simulink model "hrg_wa_compensation_research"  (R2025a)
settings: Solver=FixedStepDiscrete  StartTime=0.0  StopTime=p.duration  FixedStep=p.Ts  RelTol=1e-3
model workspace (MAT data in the model file):
  Ad = [0.987688405123  -5.68131323296e-08  2.48971225508e-05  1.72406495467e-10  2.35500029057e-16  -7.48045553179e-18  2.39085041361e-17  1.59212234261e-22  0  0  0  0; 5.68131323296e-08  0.987688405123  -1.72406495467e-10  2.48971225508e-05  4.70881019476e-18  2.69344781657e-16  -1.59212235008e-22  2.39085041361e-17  0  0  0  0; -982.899001209  -0.00680633562581  0.987672737796  1.37356342331e-05  1.5611837146e-11  -5.09714578103e-13  9.88617178136e-13  1.31942511779e-17  0  0  0  0; 0.00680633562581  -982.899001209  -1.37356342331e-05  0.987672737796  3.12106539235e-13  1.83550880441e-11  -1.31942512097e-17  9.88617178136e-13  0  0  0  0; 0  0  0  0  0.28650479686  0  0  0  0  0  0  0; 0  0  0  0  0  0.352866081459  0  0  0  0  0  0; 943869.866875  6.2854468604  -988.617130951  -0.0131942506432  -1.52887962977e-08  4.97849569843e-10  -9.75634597461e-10  -1.26518662631e-14  0  0  0  0; -6.2854468604  943869.866875  0.0131942506432  -988.617130951  -3.05654153121e-10  -1.79275916498e-08  1.26518662949e-14  -9.75634597462e-10  0  0  0  0; 113668107.931  505.246320907  -239056.237822  -1.59199430864  -2.20191905684e-06  6.98200094534e-08  9.9975990594  -1.46549020767e-12  0.999750031247  0  0  0; -505.246320907  113668107.931  1.59199430864  -239056.237822  -4.4027695682e-08  -2.51395406668e-06  1.46549021355e-12  9.9975990594  0  0.999750031247  0  0; 62170953.3395  1554505.52703  -163920.493963  -4098.88409978  -1.27454644375e-06  4.00156404796e-09  9.50410725413  0.237602681353  0.956612237767  0.0239153059442  0.0432139182638  0; -882829.706009  61193845.2426  2356.91164918  -163353.073245  -7.00440355025e-09  -1.4233603888e-06  -0.139969993764  9.70458623439  -0.0141100303999  0.97829544106  0  0.0591645112941]
  Bd = [1.07541978092e-16  -2.80909408987e-18; 2.15044631223e-18  1.01140599362e-16; 1.17750014529e-11  -3.11685647158e-13; 2.35440509738e-13  1.12226992357e-11; 0.71349520314  0; 0  0.647133918541; -1.10105605369e-08  2.90941885987e-10; -2.20157780066e-10  -1.04757152027e-08; -9.65252715165e-07  2.517993119e-08; -1.93016562843e-08  -9.06591565342e-07; -4.58609339763e-07  1.18833226824e-09; -2.49830556256e-09  -4.18846719335e-07]
  c.detect = [-9972404010.59+545538559.48i  -249313581.813+13639144.7876i; 149497357.356-9010063.9201i  -10364965233+624625194.794i]
  c.sample_period_s = 2.5e-05
  c.drive = [1.0677862215e-06-2.20398678601e-07i  -3.17521221847e-08+7.37459562675e-09i; 2.13558605901e-08-4.40799791844e-09i  1.14308593334e-06-2.65487026279e-07i]
  c.nominal_detect = -9999678898.08+46914376.8426i
  p.schema = 'v10.1'
  p.synthetic = 1
  p.f0 = 1000
  p.gamma_intrinsic = 0.314159265359
  p.Cs = 1e-09
  p.G0 = 1e-10
  p.kappa = 1e-06
  p.b = 1.1e-06
  p.Cds = 0
  p.Rs = 1000
  p.B = 0.276990961962
  p.Omega = 0.5
  p.Ts = 2.5e-05
  p.Tc = 0.001
  p.duration = 0.8
  p.charge_target = 1e-11
  p.initial_fraction = 0.3
  p.theta0 = 0.4
  p.Cf = 1e-10
  p.Rf = 1000000000
  p.driver_tau = [2e-05; 2.4e-05]
  p.afe_bw = [20000; 18000]
  p.detect_matrix = [1  0.025; -0.015  1.04]
  p.drive_matrix = [1  -0.03; 0.02  1.08]
  p.split_hz = 0
  p.stiffness_axis = 0.37
  p.damping_half_difference = 0
  p.damping_axis = -0.23
  p.adc_span = 2
  p.adc_bits = 20
  p.dac_span = 2
  p.dac_bits = 18
  p.vmax = 1
  p.agc_bw = 5
  p.quad_bw = 4
  p.pll_gain = 30
  p.max_detune = 30
  p.virtual_rate = 0
  p.virtual_start_min_s = 0.25
  p.virtual_settle_fraction = 0.01
  p.predict_heading = 1
  p.max_heading_rate = 100
  p.virtual_validated_limit = 0.2
  p.min_amplitude_fraction = 0.02
  p.min_linearity = 0.1
  p.max_calibration_condition = 100
  p.max_frame_age = 0.002
  p.calibrate_detection = 1
  p.calibrate_drive = 1
  p.noise_rms_V = 0
  p.noise_seed = 20261030
  p.heading_start_s = 0
  p.zero_start_force = 1
  p.enable_tensor_ff = 1
  p.identified_dK = [-0.00819482149803  0.00496733694019; 0.00496733694019  0.00671005445861]
  p.identified_dD = [-4.47767757243e-07  -7.60819493737e-07; -7.60819493737e-07  -1.26420490762e-06]
  x0 = [2.76318298201e-12; 1.16825502693e-12; 0; 0; 0; 0; 0; 0; 0; 0; 0; 0]
libraries: hrg_wa_v10_2_cn_modules x5
Description:
  | 条件性补偿研究：合成独立校准参考，原门限不变；20/21研究点通过不等于硬件或全工作范围认证。
settings Model: Creator=11725  LastModifiedBy=11725

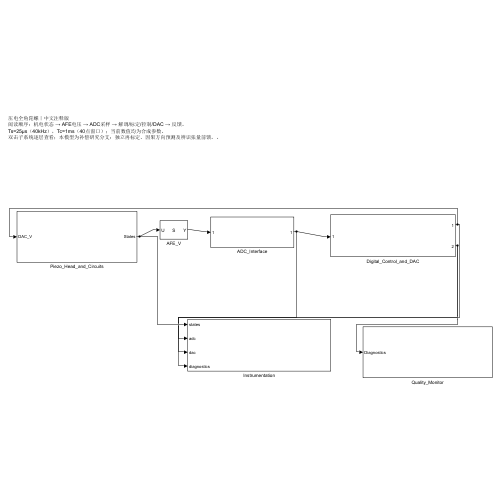
[thumbnail: Simulink's stored preview of the top-level diagram]
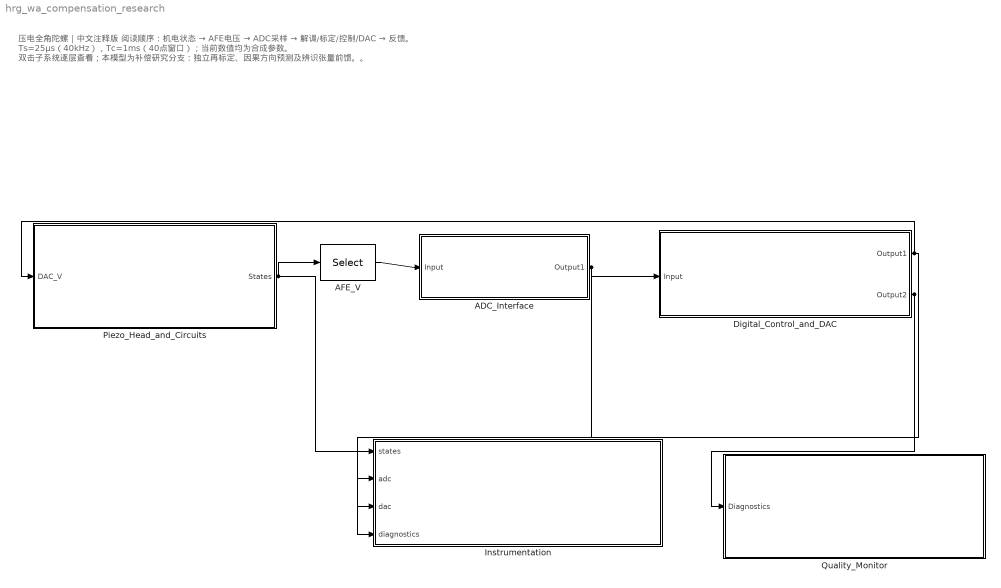
== system hrg_wa_compensation_research ==
  note: 压电全角陀螺｜中文注释版
      | 阅读顺序：机电状态 → AFE电压 → ADC采样 → 解调/标定/控制/DAC → 反馈。
      | Ts=25μs（40kHz），Tc=1ms（40点窗口）；当前数值均为合成参数。
      | 双击子系统逐层查看；本模型为补偿研究分支：独立再标定、因果方向预测及辨识张量前馈。。
  ADC_Interface : Subsystem  Description=输入噪声、ADC整数码量化与两路截幅标志；详见pcn_adc_sfun.m及pcn_quantize.m。
  AFE_V : Selector  InputPortWidth=12  IndexOptions=Index vector (dialog)  Indices=[11 12]  OutputSizes=1
  Digital_Control_and_DAC : Subsystem  Description=补偿研究内核comp_tick：从有效测量开始因果方向预测，首帧前零力；独立辨识ΔK/ΔD前馈。控制不读取真实Omega或机械各向异性真值。
  Instrumentation : Subsystem  Description=14个Scope、2个频谱仪和4组To Workspace；角度评分见pcn_metrics.m。
  Piezo_Head_and_Circuits : Subsystem  Description=压电表头及电路的联合离散模型；五个库模块共12个状态，端口输出顺序见画布。
  Quality_Monitor : Subsystem
  wires:
  Piezo_Head_and_Circuits/1(States) -> AFE_V/1, Instrumentation/1(states)
  AFE_V/1 -> ADC_Interface/1(Input)
  ADC_Interface/1(Output1) -> Digital_Control_and_DAC/1(Input), Instrumentation/2(adc)
  Digital_Control_and_DAC/1(Output1) -> Piezo_Head_and_Circuits/1(DAC_V), Instrumentation/3(dac)
  Digital_Control_and_DAC/2(Output2) -> Instrumentation/4(diagnostics), Quality_Monitor/1(Diagnostics)

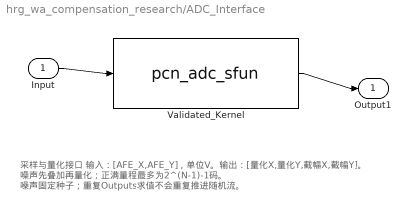
== system hrg_wa_compensation_research/ADC_Interface ==
  note: 采样与量化接口
      | 输入：[AFE_X,AFE_Y]，单位V。输出：[量化X,量化Y,截幅X,截幅Y]。
      | 噪声先叠加再量化；正满量程最多为2^(N-1)-1码。
      | 噪声固定种子；重复Outputs求值不会重复推进随机流。
  Input : Inport
  Validated_Kernel : M-S-Function  FunctionName=pcn_adc_sfun  Parameters=p
  Output1 : Outport
  wires:
  Input/1 -> Validated_Kernel/1
  Validated_Kernel/1 -> Output1/1

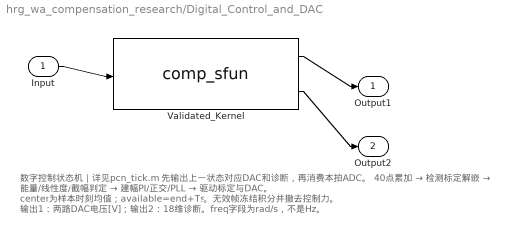
== system hrg_wa_compensation_research/Digital_Control_and_DAC ==
  note: 数字控制状态机｜详见pcn_tick.m
      | 先输出上一状态对应DAC和诊断，再消费本拍ADC。
      | 40点累加 → 检测标定解嵌 → 能量/线性度/截幅判定 → 建幅PI/正交/PLL → 驱动标定与DAC。
      | center为样本时刻均值；available=end+Ts。无效帧冻结积分并撤去控制力。
      | 输出1：两路DAC电压[V]；输出2：18维诊断。freq字段为rad/s，不是Hz。
  Input : Inport
  Validated_Kernel : M-S-Function  Description=comp_sfun调用comp_tick，35维状态不变；前馈为(identified_dK+jω identified_dD)*(I-jQ)，主轴固定在表头坐标。  FunctionName=comp_sfun  Parameters=p,c
  Output1 : Outport
  Output2 : Outport  Port=2
  wires:
  Input/1 -> Validated_Kernel/1
  Validated_Kernel/1 -> Output1/1
  Validated_Kernel/2 -> Output2/1

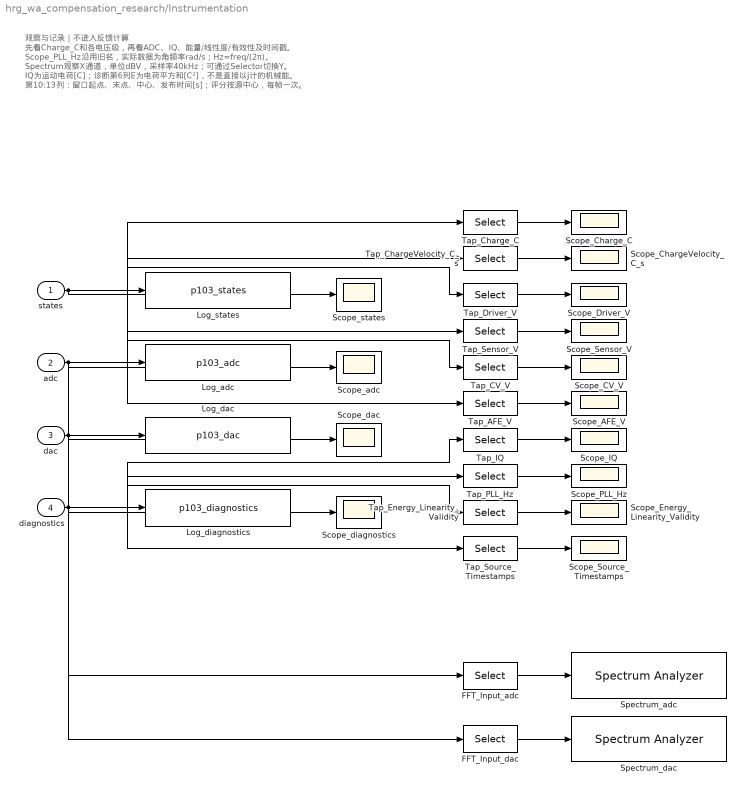
== system hrg_wa_compensation_research/Instrumentation ==
  note: 观察与记录｜不进入反馈计算
      | 先看Charge_C和各电压级，再看ADC、IQ、能量/线性度/有效性及时间戳。
      | Scope_PLL_Hz沿用旧名，实际数据为角频率rad/s；Hz=freq/(2π)。
      | Spectrum观察X通道，单位dBV，采样率40kHz；可通过Selector切换Y。
      | IQ为运动电荷[C]；诊断第6列E为电荷平方和[C²]，不是直接以J计的机械能。
      | 第10:13列：窗口起点、末点、中心、发布时间[s]；评分按源中心，每帧一次。
  states : Inport
  adc : Inport  Port=2
  dac : Inport  Port=3
  diagnostics : Inport  Port=4
  FFT_Input_adc : Selector  InputPortWidth=4  IndexOptions=Index vector (dialog)  Indices=1  OutputSizes=1
  FFT_Input_dac : Selector  InputPortWidth=2  IndexOptions=Index vector (dialog)  Indices=1  OutputSizes=1
  Log_adc : ToWorkspace  VariableName=p103_adc  SaveFormat=Timeseries  SampleTime=-1
  Log_dac : ToWorkspace  VariableName=p103_dac  SaveFormat=Timeseries  SampleTime=-1
  Log_diagnostics : ToWorkspace  VariableName=p103_diagnostics  SaveFormat=Timeseries  SampleTime=-1
  Log_states : ToWorkspace  VariableName=p103_states  SaveFormat=Timeseries  SampleTime=-1
  Scope_AFE_V : Scope
  Scope_CV_V : Scope
  Scope_ChargeVelocity_C_s : Scope
  Scope_Charge_C : Scope
  Scope_Driver_V : Scope
  Scope_Energy_Linearity_Validity : Scope
  Scope_IQ : Scope
  Scope_PLL_Hz : Scope
  Scope_Sensor_V : Scope
  Scope_Source_Timestamps : Scope
  Scope_adc : Scope
  Scope_dac : Scope
  Scope_diagnostics : Scope
  Scope_states : Scope
  Spectrum_adc : SpectrumAnalyzer  SampleRateSource=Property  SampleRate=1/p.Ts  WindowInvariantSamplesPerUpdate=on  SpectrumUnits=dBV
      settings: OpenAtSimulationStart=off
  Spectrum_dac : SpectrumAnalyzer  SampleRateSource=Property  SampleRate=1/p.Ts  WindowInvariantSamplesPerUpdate=on  SpectrumUnits=dBV
      settings: OpenAtSimulationStart=off
  Tap_AFE_V : Selector  InputPortWidth=12  IndexOptions=Index vector (dialog)  Indices=[11 12]  OutputSizes=1
  Tap_CV_V : Selector  InputPortWidth=12  IndexOptions=Index vector (dialog)  Indices=[9 10]  OutputSizes=1
  Tap_ChargeVelocity_C_s : Selector  InputPortWidth=12  IndexOptions=Index vector (dialog)  Indices=[3 4]  OutputSizes=1
  Tap_Charge_C : Selector  InputPortWidth=12  IndexOptions=Index vector (dialog)  Indices=[1 2]  OutputSizes=1
  Tap_Driver_V : Selector  InputPortWidth=12  IndexOptions=Index vector (dialog)  Indices=[5 6]  OutputSizes=1
  Tap_Energy_Linearity_Validity : Selector  InputPortWidth=18  IndexOptions=Index vector (dialog)  Indices=[6 7 8]  OutputSizes=1
  Tap_IQ : Selector  InputPortWidth=18  IndexOptions=Index vector (dialog)  Indices=[1 2 3 4]  OutputSizes=1
  Tap_PLL_Hz : Selector  InputPortWidth=18  IndexOptions=Index vector (dialog)  Indices=5  OutputSizes=1
  Tap_Sensor_V : Selector  InputPortWidth=12  IndexOptions=Index vector (dialog)  Indices=[7 8]  OutputSizes=1
  Tap_Source_Timestamps : Selector  InputPortWidth=18  IndexOptions=Index vector (dialog)  Indices=[10 11 12 13]  OutputSizes=1
  wires:
  states/1 -> Log_states/1, Scope_states/1, Tap_Charge_C/1, Tap_ChargeVelocity_C_s/1, Tap_Driver_V/1, Tap_Sensor_V/1, Tap_CV_V/1, Tap_AFE_V/1
  adc/1 -> Log_adc/1, Scope_adc/1, FFT_Input_adc/1
  dac/1 -> Log_dac/1, Scope_dac/1, FFT_Input_dac/1
  diagnostics/1 -> Log_diagnostics/1, Scope_diagnostics/1, Tap_IQ/1, Tap_PLL_Hz/1, Tap_Energy_Linearity_Validity/1, Tap_Source_Timestamps/1
  Tap_Charge_C/1 -> Scope_Charge_C/1
  Tap_ChargeVelocity_C_s/1 -> Scope_ChargeVelocity_C_s/1
  Tap_Driver_V/1 -> Scope_Driver_V/1
  Tap_Sensor_V/1 -> Scope_Sensor_V/1
  Tap_CV_V/1 -> Scope_CV_V/1
  Tap_AFE_V/1 -> Scope_AFE_V/1
  Tap_IQ/1 -> Scope_IQ/1
  Tap_PLL_Hz/1 -> Scope_PLL_Hz/1
  Tap_Energy_Linearity_Validity/1 -> Scope_Energy_Linearity_Validity/1
  Tap_Source_Timestamps/1 -> Scope_Source_Timestamps/1
  FFT_Input_adc/1 -> Spectrum_adc/1
  FFT_Input_dac/1 -> Spectrum_dac/1

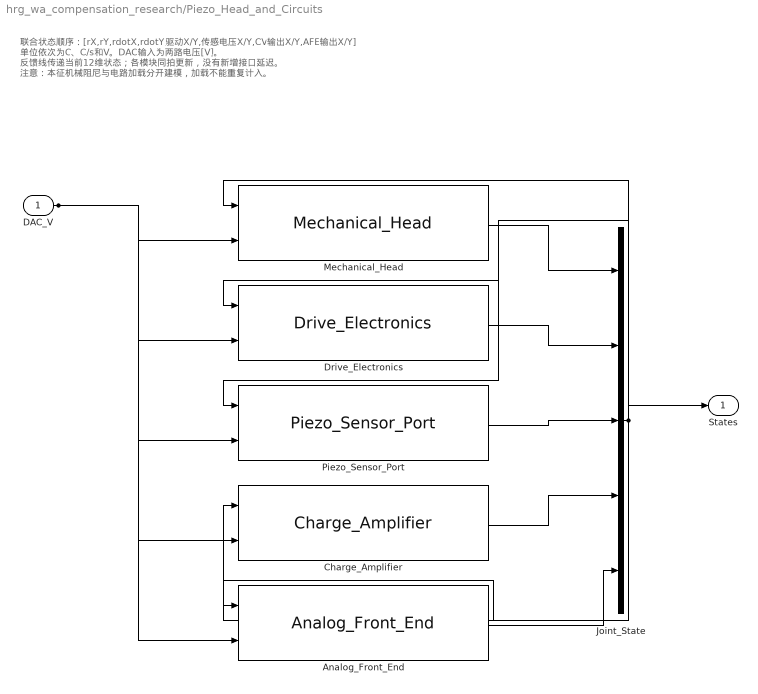
== system hrg_wa_compensation_research/Piezo_Head_and_Circuits ==
  note: 联合状态顺序：[rX,rY,rdotX,rdotY,驱动X/Y,传感电压X/Y,CV输出X/Y,AFE输出X/Y]
      | 单位依次为C、C/s和V。DAC输入为两路电压[V]。
      | 反馈线传递当前12维状态；各模块同拍更新，没有新增接口延迟。
      | 注意：本征机械阻尼与电路加载分开建模，加载不能重复计入。
  DAC_V : Inport
  Analog_Front_End : hrg_wa_v10_2_cn_modules/Analog_Front_End  Description=|  SystemSampleTime=-1  VariantActivationTime=update diagram  EmptyChoice=off  PassThrough=off  PassThroughVariantControl=(default)  EmptyChoiceVariantControl=(default)  AllowFlexibleInterface=on  Latency=0  AutoFrameSizeCalculation=off
      | 模拟前端AFE｜带宽及通道耦合
      | 状态11:12为ADC前电压[V]。afe_bw为Hz，内部乘2π换成角频率。
      | 检测矩阵包含两通道幅值不一致与串扰。
  Charge_Amplifier : hrg_wa_v10_2_cn_modules/Charge_Amplifier  Description=|  SystemSampleTime=-1  VariantActivationTime=update diagram  EmptyChoice=off  PassThrough=off  PassThroughVariantControl=(default)  EmptyChoiceVariantControl=(default)  AllowFlexibleInterface=on  Latency=0  AutoFrameSizeCalculation=off
      | 电荷放大器｜积分及泄放
      | 状态9:10为输出电压[V]。Cf决定电荷/电压增益，Rf提供直流泄放。
      | 输出还需经过AFE，不能直接当作理想运动电荷。
  Drive_Electronics : hrg_wa_v10_2_cn_modules/Drive_Electronics  Description=|  SystemSampleTime=-1  VariantActivationTime=update diagram  EmptyChoice=off  PassThrough=off  PassThroughVariantControl=(default)  EmptyChoiceVariantControl=(default)  AllowFlexibleInterface=on  Latency=0  AutoFrameSizeCalculation=off
      | 驱动电子学｜双通道一阶带宽
      | 状态5:6为驱动器电压[V]。DAC输入为两路采样电压[V]。
      | 通道时间常数driver_tau及drive_matrix描述不一致与串扰。
  Joint_State : Mux  Inputs=5
  Mechanical_Head : hrg_wa_v10_2_cn_modules/Mechanical_Head  Description=|  SystemSampleTime=-1  VariantActivationTime=update diagram  EmptyChoice=off  PassThrough=off  PassThroughVariantControl=(default)  EmptyChoiceVariantControl=(default)  AllowFlexibleInterface=on  Latency=0  AutoFrameSizeCalculation=off
      | 机械表头｜二维二阶模态
      | 状态1:2为运动电荷r[C]，3:4为电荷速度[C/s]。
      | 刚度、阻尼可有不同主轴；角速度经科里奥利项耦合。
      | 输入是当前联合12维状态和DAC电压，不是独立机械力接口。
  Piezo_Sensor_Port : hrg_wa_v10_2_cn_modules/Piezo_Sensor_Port  Description=|  SystemSampleTime=-1  VariantActivationTime=update diagram  EmptyChoice=off  PassThrough=off  PassThroughVariantControl=(default)  EmptyChoiceVariantControl=(default)  AllowFlexibleInterface=on  Latency=0  AutoFrameSizeCalculation=off
      | 压电传感端口｜互易机电加载
      | 状态7:8为节点电压[V]。Cs、G0、Rs及运动电荷电流共同作用。
      | 端口电压回作用机械运动；不可把加载衰减率再次加到本征阻尼。
  States : Outport
  wires:
  Joint_State/1 -> Mechanical_Head/1, Drive_Electronics/1, Piezo_Sensor_Port/1, Charge_Amplifier/1, Analog_Front_End/1, States/1
  DAC_V/1 -> Mechanical_Head/2, Drive_Electronics/2, Piezo_Sensor_Port/2, Charge_Amplifier/2, Analog_Front_End/2
  Mechanical_Head/1 -> Joint_State/1
  Drive_Electronics/1 -> Joint_State/2
  Piezo_Sensor_Port/1 -> Joint_State/3
  Charge_Amplifier/1 -> Joint_State/4
  Analog_Front_End/1 -> Joint_State/5

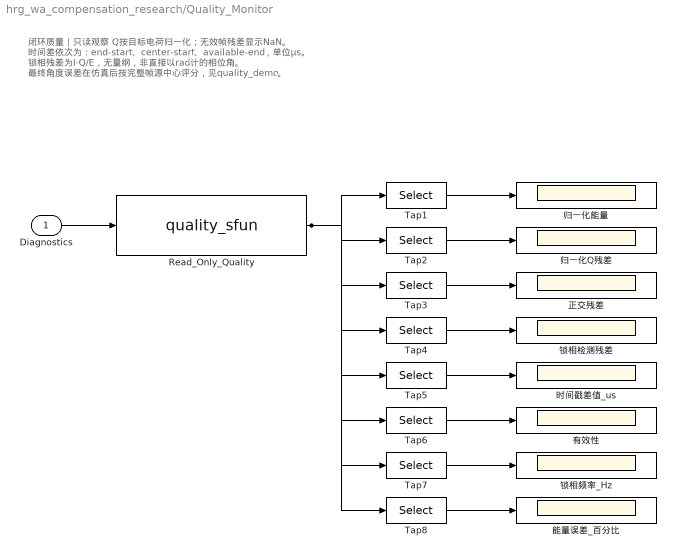
== system hrg_wa_compensation_research/Quality_Monitor ==
  note: 闭环质量｜只读观察
      | Q按目标电荷归一化；无效帧残差显示NaN。
      | 时间差依次为：end-start、center-start、available-end，单位μs。
      | 锁相残差为I·Q/E，无量纲，非直接以rad计的相位角。
      | 最终角度误差在仿真后按完整帧源中心评分，见quality_demo。
  Diagnostics : Inport
  Read_Only_Quality : M-S-Function  FunctionName=quality_sfun  Parameters=p
  Tap1 : Selector  InputPortWidth=11  IndexOptions=Index vector (dialog)  Indices=1  OutputSizes=1
  Tap2 : Selector  InputPortWidth=11  IndexOptions=Index vector (dialog)  Indices=[2 3]  OutputSizes=1
  Tap3 : Selector  InputPortWidth=11  IndexOptions=Index vector (dialog)  Indices=4  OutputSizes=1
  Tap4 : Selector  InputPortWidth=11  IndexOptions=Index vector (dialog)  Indices=5  OutputSizes=1
  Tap5 : Selector  InputPortWidth=11  IndexOptions=Index vector (dialog)  Indices=[6 7 8]  OutputSizes=1
  Tap6 : Selector  InputPortWidth=11  IndexOptions=Index vector (dialog)  Indices=9  OutputSizes=1
  Tap7 : Selector  InputPortWidth=11  IndexOptions=Index vector (dialog)  Indices=10  OutputSizes=1
  Tap8 : Selector  InputPortWidth=11  IndexOptions=Index vector (dialog)  Indices=11  OutputSizes=1
  归一化Q残差 : Scope
  归一化能量 : Scope
  时间戳差值_us : Scope
  有效性 : Scope
  正交残差 : Scope
  能量误差_百分比 : Scope
  锁相检测残差 : Scope
  锁相频率_Hz : Scope
  wires:
  Diagnostics/1 -> Read_Only_Quality/1
  Read_Only_Quality/1 -> Tap1/1, Tap2/1, Tap3/1, Tap4/1, Tap5/1, Tap6/1, Tap7/1, Tap8/1
  Tap1/1 -> 归一化能量/1
  Tap2/1 -> 归一化Q残差/1
  Tap3/1 -> 正交残差/1
  Tap4/1 -> 锁相检测残差/1
  Tap5/1 -> 时间戳差值_us/1
  Tap6/1 -> 有效性/1
  Tap7/1 -> 锁相频率_Hz/1
  Tap8/1 -> 能量误差_百分比/1
